simulink model "Cell_Balancer_V_2"  (R2026b)
settings: Solver=VariableStepAuto  StopTime=72000
InitFcn:
  | R=4.2
  | A=.2
  | B=.25
  | C=.24
  | D=.23
  | E=.29
  | F=.22
  | G=.26
  | H=.27
  | I=.28
  | J=.21
libraries: fl_lib x43, nesl_utility x33, batt_lib x10, BatteryCurrentManagement x1
(part 4 of 4)

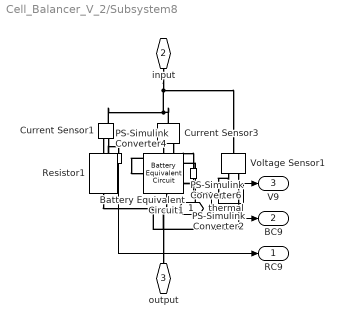
== system Cell_Balancer_V_2/Subsystem8 ==
  Battery Equivalent Circuit1 : batt_lib/Cells/Battery Equivalent Circuit  BatteryCapacity=3 A*hr  ThermalModel=simscape.battery.enum.cells.BatteryThermalModel.LumpedThermalMass  ExtrapolationMethod=simscape.enum.extrapolation.nearest  SOCBreakpoints=[0, .1, .25, .5, .75, .9, 1]  TemperatureBreakpoints=[278, 293, 313] K  OpenCircuitVoltage=[3.5057, 3.566, 3.6337, 3.7127, 3.9259, 4.0777, 4.1928] V  OpenCircuitVoltageThermal=|  VoltageRange=[0, inf] V  HysteresisModel=simscape.battery.enum.cells.HysteresisModel.none  MaximumHysteresisVoltage=[0, 0, 0, 0, 0, 0, 0] V  InstantaneousHysteresisVoltage=[0, 0, 0, 0, 0, 0, 0] V  HysteresisRate=0.1  MaximumHysteresisVoltageThermal=[0, 0, 0; 0, 0, 0; 0, 0, 0; 0, 0, 0; 0, 0, 0; 0, 0, 0; 0, 0, 0] V  InstantaneousHysteresisVoltageThermal=[0, 0, 0; 0, 0, 0; 0, 0, 0; 0, 0, 0; 0, 0, 0; 0, 0, 0; 0, 0, 0] V  HysteresisRateThermal=0.1  ResistanceSOCBreakpoints=[0, .1, .25, .5, .75, .9, 1]  ResistanceTemperatureBreakpoints=[278, 293, 313] K  ResistanceCurrentBreakpoints=[-1, 0, 1] A  CurrentDependence=simscape.battery.enum.cells.CurrentDependence.Disabled  R0=[.0085, .0085, .0087, .0082, .0083, .0085, .0085] Ohm  R0I=[.0117, .0085, .009; .011, .0085, .009; .0114, .0087, .0092; .0107, .0082, .0088; .0107, .0083, .0091; .0113, .0085, .0089; .0116, .0085, .0089] Ohm  R0Thermal=[.0117, .0085, .009; .011, .0085, .009; .0114, .0087, .0092; .0107, .0082, .0088; .0107, .0083, .0091; .0113, .0085, .0089; .0116, .0085, .0089] Ohm  R0ThermalI=repmat([.0117, .0085, .009; .011, .0085, .009; .0114, .0087, .0092; .0107, .0082, .0088; .0107, .0083, .0091; .0113, .0085, .0089; .0116, .0085, .0089], 1, 1, 3) Ohm  DischargeR0=[.0085, .0085, .0087, .0082, .0083, .0085, .0085] Ohm  ChargeR0=[.0085, .0085, .0087, .0082, .0083, .0085, .0085] Ohm  ChargeR0Thermal=[.0117, .0085, .009; .011, .0085, .009; .0114, .0087, .0092; .0107, .0082, .0088; .0107, .0083, .0091; .0113, .0085, .0089; .0116, .0085, .0089] Ohm  DischargeR0Thermal=[.0117, .0085, .009; .011, .0085, .009; .0114, .0087, .0092; .0107, .0082, .0088; .0107, .0083, .0091; .0113, .0085, .0089; .0116, .0085, .0089] Ohm  RCPairs=simscape.battery.enum.cells.RCPairs.noDynamics  R1=[.0029, .0024, .0026, .0016, .0023, .0018, .0017] Ohm  Tau1=[36, 45, 105, 29, 77, 33, 39] s  R2=[.0029, .0024, .0026, .0016, .0023, .0018, .0017] Ohm  Tau2=[36, 45, 105, 29, 77, 33, 39] s  R3=[.0029, .0024, .0026, .0016, .0023, .0018, .0017] Ohm  Tau3=[36, 45, 105, 29, 77, 33, 39] s  R1I=[.0109, .0029, .0013; .0069, .0024, .0012; .0047, .0026, .0013; .0034, .0016, .001; .0033, .0023, .0014; .0033, .0018, .0011; .0028, .0017, .0011] Ohm  Tau1I=[20, 36, 39; 31, 45, 39; 109, 105, 61; 36, 29, 26; 59, 77, 67; 40, 33, 29; 25, 39, 33] s  R2I=[.0109, .0029, .0013; .0069, .0024, .0012; .0047, .0026, .0013; .0034, .0016, .001; .0033, .0023, .0014; .0033, .0018, .0011; .0028, .0017, .0011] Ohm  Tau2I=[20, 36, 39; 31, 45, 39; 109, 105, 61; 36, 29, 26; 59, 77, 67; 40, 33, 29; 25, 39, 33] s  R3I=[.0109, .0029, .0013; .0069, .0024, .0012; .0047, .0026, .0013; .0034, .0016, .001; .0033, .0023, .0014; .0033, .0018, .0011; .0028, .0017, .0011] Ohm  Tau3I=[20, 36, 39; 31, 45, 39; 109, 105, 61; 36, 29, 26; 59, 77, 67; 40, 33, 29; 25, 39, 33] s  DischargeR1=[.0029, .0024, .0026, .0016, .0023, .0018, .0017] Ohm  DischargeTau1=[36, 45, 105, 29, 77, 33, 39] s  ChargeR1=[.0029, .0024, .0026, .0016, .0023, .0018, .0017] Ohm  ChargeTau1=[36, 45, 105, 29, 77, 33, 39] s  DischargeR2=[.0029, .0024, .0026, .0016, .0023, .0018, .0017] Ohm  DischargeTau2=[36, 45, 105, 29, 77, 33, 39] s  ChargeR2=[.0029, .0024, .0026, .0016, .0023, .0018, .0017] Ohm  ChargeTau2=[36, 45, 105, 29, 77, 33, 39] s  DischargeR3=[.0029, .0024, .0026, .0016, .0023, .0018, .0017] Ohm  DischargeTau3=[36, 45, 105, 29, 77, 33, 39] s  ChargeR3=[.0029, .0024, .0026, .0016, .0023, .0018, .0017] Ohm  ChargeTau3=[36, 45, 105, 29, 77, 33, 39] s  R1Thermal=[.0109, .0029, .0013; .0069, .0024, .0012; .0047, .0026, .0013; .0034, .0016, .001; .0033, .0023, .0014; .0033, .0018, .0011; .0028, .0017, .0011] Ohm  Tau1Thermal=[20, 36, 39; 31, 45, 39; 109, 105, 61; 36, 29, 26; 59, 77, 67; 40, 33, 29; 25, 39, 33] s  R2Thermal=[.0109, .0029, .0013; .0069, .0024, .0012; .0047, .0026, .0013; .0034, .0016, .001; .0033, .0023, .0014; .0033, .0018, .0011; .0028, .0017, .0011] Ohm  Tau2Thermal=[20, 36, 39; 31, 45, 39; 109, 105, 61; 36, 29, 26; 59, 77, 67; 40, 33, 29; 25, 39, 33] s  R3Thermal=[.0109, .0029, .0013; .0069, .0024, .0012; .0047, .0026, .0013; .0034, .0016, .001; .0033, .0023, .0014; .0033, .0018, .0011; .0028, .0017, .0011] Ohm  Tau3Thermal=[20, 36, 39; 31, 45, 39; 109, 105, 61; 36, 29, 26; 59, 77, 67; 40, 33, 29; 25, 39, 33] s  R1ThermalI=repmat([.0109, .0029, .0013; .0069, .0024, .0012; .0047, .0026, .0013; .0034, .0016, .001; .0033, .0023, .0014; .0033, .0018, .0011; .0028, .0017, .0011], 1, 1, 3) Ohm  Tau1ThermalI=repmat([20, 36, 39; 31, 45, 39; 109, 105, 61; 36, 29, 26; 59, 77, 67; 40, 33, 29; 25, 39, 33], 1, 1, 3) s  R2ThermalI=repmat([.0109, .0029, .0013; .0069, .0024, .0012; .0047, .0026, .0013; .0034, .0016, .001; .0033, .0023, .0014; .0033, .0018, .0011; .0028, .0017, .0011], 1, 1, 3) Ohm  Tau2ThermalI=repmat([20, 36, 39; 31, 45, 39; 109, 105, 61; 36, 29, 26; 59, 77, 67; 40, 33, 29; 25, 39, 33], 1, 1, 3) s  R3ThermalI=repmat([.0109, .0029, .0013; .0069, .0024, .0012; .0047, .0026, .0013; .0034, .0016, .001; .0033, .0023, .0014; .0033, .0018, .0011; .0028, .0017, .0011], 1, 1, 3) Ohm  Tau3ThermalI=repmat([20, 36, 39; 31, 45, 39; 109, 105, 61; 36, 29, 26; 59, 77, 67; 40, 33, 29; 25, 39, 33], 1, 1, 3) s  DischargeR1Thermal=[.0109, .0029, .0013; .0069, .0024, .0012; .0047, .0026, .0013; .0034, .0016, .001; .0033, .0023, .0014; .0033, .0018, .0011; .0028, .0017, .0011] Ohm  DischargeTau1Thermal=[20, 36, 39; 31, 45, 39; 109, 105, 61; 36, 29, 26; 59, 77, 67; 40, 33, 29; 25, 39, 33] s  ChargeR1Thermal=[.0109, .0029, .0013; .0069, .0024, .0012; .0047, .0026, .0013; .0034, .0016, .001; .0033, .0023, .0014; .0033, .0018, .0011; .0028, .0017, .0011] Ohm  ChargeTau1Thermal=[20, 36, 39; 31, 45, 39; 109, 105, 61; 36, 29, 26; 59, 77, 67; 40, 33, 29; 25, 39, 33] s  DischargeR2Thermal=[.0109, .0029, .0013; .0069, .0024, .0012; .0047, .0026, .0013; .0034, .0016, .001; .0033, .0023, .0014; .0033, .0018, .0011; .0028, .0017, .0011] Ohm  DischargeTau2Thermal=[20, 36, 39; 31, 45, 39; 109, 105, 61; 36, 29, 26; 59, 77, 67; 40, 33, 29; 25, 39, 33] s  ChargeR2Thermal=[.0109, .0029, .0013; .0069, .0024, .0012; .0047, .0026, .0013; .0034, .0016, .001; .0033, .0023, .0014; .0033, .0018, .0011; .0028, .0017, .0011] Ohm  ChargeTau2Thermal=[20, 36, 39; 31, 45, 39; 109, 105, 61; 36, 29, 26; 59, 77, 67; 40, 33, 29; 25, 39, 33] s  DischargeR3Thermal=[.0109, .0029, .0013; .0069, .0024, .0012; .0047, .0026, .0013; .0034, .0016, .001; .0033, .0023, .0014; .0033, .0018, .0011; .0028, .0017, .0011] Ohm  DischargeTau3Thermal=[20, 36, 39; 31, 45, 39; 109, 105, 61; 36, 29, 26; 59, 77, 67; 40, 33, 29; 25, 39, 33] s  ChargeR3Thermal=[.0109, .0029, .0013; .0069, .0024, .0012; .0047, .0026, .0013; .0034, .0016, .001; .0033, .0023, .0014; .0033, .0018, .0011; .0028, .0017, .0011] Ohm  ChargeTau3Thermal=[20, 36, 39; 31, 45, 39; 109, 105, 61; 36, 29, 26; 59, 77, 67; 40, 33, 29; 25, 39, 33] s  SelfDischargeResistor=simscape.battery.enum.cells.BatteryEnable.Disabled  SelfDischargeR=7e3 Ohm  SelfDischargeRThermal=[8000, 7000, 6000] Ohm  CyclingAgingMethod=simscape.battery.enum.cells.CyclingAgingMethod.disabled  CycleCalculationMethod=simscape.battery.enum.cells.CycleCalculationMethod.EquivalentCycles  NumDisCycles=100  OCVChange=0  R0Change=0  CapacityChange=0  SelfDischargeRChange=0  R1Change=0  R2Change=0  R3Change=0  NumDisCyclesBreakpoints=[0, 100, 200, 300]  AgingTemperatureBreakpoints=[298.15, 323.15] K  AgingCurrentBreakpoints=[-.1, -.5, -5] A  OCVChangeVec=[0, 0, 0, 0]  OCVChangeThermal=[0, 0; 0, 0; 0, 0; 0, 0]  R0ChangeVec=[0, 0, 0, 0]  R0ChangeThermal=[0, 0; 0, 0; 0, 0; 0, 0]  R0ChangeThermalI=repmat(0, 4, 2, 3)  R0CyclingChangeInitialTarget=0  CapacityChangeVec=[0, 0, 0, 0]  CapacityChangeThermal=[0, 0; 0, 0; 0, 0; 0, 0]  CapacityChangeThermalI=repmat(0, 4, 2, 3)  CapacityCyclingChangeInitialTarget=0  SelfDischargeRChangeVec=[0, 0, 0, 0]  SelfDischargeRChangeThermal=[0, 0; 0, 0; 0, 0; 0, 0]  SelfDischargeRChangeThermalI=repmat(0, 4, 2, 3)  SelfDischargeRCyclingChangeInitialTarget=0  R1ChangeVec=[0, 0, 0, 0]  R1ChangeThermal=[0, 0; 0, 0; 0, 0; 0, 0]  R1ChangeThermalI=repmat(0, 4, 2, 3)  R1CyclingChangeInitialTarget=0  R2ChangeVec=[0, 0, 0, 0]  R2ChangeThermal=[0, 0; 0, 0; 0, 0; 0, 0]  R2ChangeThermalI=repmat(0, 4, 2, 3)  R2CyclingChangeInitialTarget=0  R3ChangeVec=[0, 0, 0, 0]  R3ChangeThermal=[0, 0; 0, 0; 0, 0; 0, 0]  R3ChangeThermalI=repmat(0, 4, 2, 3)  R3CyclingChangeInitialTarget=0  CalendarAgeResistance=simscape.battery.enum.cells.BatteryEnable.Disabled  CalendarAgeCapacity=simscape.battery.enum.cells.BatteryEnable.Disabled  CalendarAgingMethod=simscape.battery.enum.cells.CalendarAgingMethod.equation  StorageVariable=simscape.battery.enum.cells.StorageVariable.OCV  OCVDuringStorage=0.9  SOCDuringStorage=0.6  StorageTimeIntervals=[0] d  StorageTemperatures=[273] K  ResistanceScalingOCV=2.2134e6  ResistanceScalingOCVOffset=1.632e6  ResistanceExponentialIncrease=0.515833569 V  ResistanceTimeExponent=0.75  ResistanceAgeTemperatureBreakpoints=[273.15, 298.15, 323.15] K  ResistanceAgeTimeBreakpoints=[0, 90, 180, 270] d  PercentResistanceChange=[0, 0, 0]  ResistanceTimeBreakpoints=100 d  PercentResistanceChangeThermal=[0, 0, 0; 0, 0, 0; 0, 0, 0; 0, 0, 0]  CapacityScalingOCV=1.5097e07  CapacityScalingOCVOffset=8.3625e06  CapacityExponentialIncrease=0.6011 V  CapacityTimeExponent=0.75  CapacityAgeTemperatureBreakpoints=[273.15, 298.15, 323.15] K  CapacityAgeTimeBreakpoints=[0, 90, 180, 270] d  PercentCapacityChange=[0, 0, 0]  CapacityTimeBreakpoints=100 d  PercentCapacityChangeThermal=[0, 0, 0; 0, 0, 0; 0, 0, 0; 0, 0, 0]  SimulationTemperature=298.15 K  BatteryThermalMass=100 J/K  NumThermalModels=6  ThermalConductivityZ=18 W/(K*m)  CrossSectionalAreaXY=3.5e-4 m^2  Height=0.07 m  ReversibleHeatModel=simscape.battery.enum.cells.ReversibleHeatModel.Disabled  EntropicCoefficient=[0, 0, 0, 0, 0, 0, 0] mV/K  CurrentDirectionality=simscape.battery.enum.cells.BatteryEnable.Disabled  stateOfCharge_specify=on  stateOfCharge_priority=High  stateOfCharge=I  stateOfCharge_nominal_specify=off  stateOfCharge_nominal_value=1  stateOfCharge_nominal_unit=1  batteryVoltage_specify=off  batteryVoltage_priority=None  batteryVoltage=0 V  batteryVoltage_nominal_specify=off  batteryVoltage_nominal_value=1  batteryVoltage_nominal_unit=V  batteryCurrent_specify=off  batteryCurrent_priority=None  batteryCurrent=0 A  batteryCurrent_nominal_specify=off  batteryCurrent_nominal_value=1  batteryCurrent_nominal_unit=A  numCycles_specify=off  numCycles_priority=High  numCycles=0  numCycles_nominal_specify=off  numCycles_nominal_value=1  numCycles_nominal_unit=1  batteryTemperature_specify=off  batteryTemperature_priority=High  batteryTemperature=298.15 K  batteryTemperature_nominal_specify=off  batteryTemperature_nominal_value=1  batteryTemperature_nominal_unit=K  hysteresisState_specify=off  hysteresisState_priority=High  hysteresisState=0  hysteresisState_nominal_specify=off  hysteresisState_nominal_value=1  hysteresisState_nominal_unit=1  isExothermFaulted_specify=off  isExothermFaulted_priority=None  isExothermFaulted=0  isExothermFaulted_nominal_specify=off  isExothermFaulted_nominal_value=1  isExothermFaulted_nominal_unit=1  reactionHeatRate_specify=off  reactionHeatRate_priority=None  reactionHeatRate=0 W  reactionHeatRate_nominal_specify=off  reactionHeatRate_nominal_value=1  reactionHeatRate_nominal_unit=W  reactionExtent_specify=off  reactionExtent_priority=None  reactionExtent=0  reactionExtent_nominal_specify=off  reactionExtent_nominal_value=1  reactionExtent_nominal_unit=1  shortResistorPower_specify=off  shortResistorPower_priority=None  shortResistorPower=0 W  shortResistorPower_nominal_specify=off  shortResistorPower_nominal_value=1  shortResistorPower_nominal_unit=W
      | [
      |     2.50  2.51  2.52
      |     2.78  2.79  2.80
      |     3.07  3.08  3.09
      |     3.35  3.36  3.37
      |     3.63  3.64  3.65
      |     3.91  3.92  3.93
      |     4.20  4.21  4.22
      | ]
      |  V
  Current Sensor1 : fl_lib/Electrical/Electrical Sensors/Current Sensor
  Current Sensor3 : fl_lib/Electrical/Electrical Sensors/Current Sensor
  PS-Simulink Converter2 : nesl_utility/PS-Simulink Converter  PhysicalDomain=network_engine_domain  SubClassName=ps_output  LeftPortType=input  RightPortType=output  PseudoPeriodic=off  Frequencies=[]  VectorFormat=inherit  Unit=inherit  AffineConversion=off
  PS-Simulink Converter4 : nesl_utility/PS-Simulink Converter  PhysicalDomain=network_engine_domain  SubClassName=ps_output  LeftPortType=input  RightPortType=output  PseudoPeriodic=off  Frequencies=[]  VectorFormat=inherit  Unit=inherit  AffineConversion=off
  PS-Simulink Converter6 : nesl_utility/PS-Simulink Converter  PhysicalDomain=network_engine_domain  SubClassName=ps_output  LeftPortType=input  RightPortType=output  PseudoPeriodic=off  Frequencies=[]  VectorFormat=inherit  Unit=inherit  AffineConversion=off
  Resistor1 : fl_lib/Electrical/Electrical Elements/Resistor  R=R Ohm  i_specify=off  i_priority=None  i=0 A  i_nominal_specify=off  i_nominal_value=1  i_nominal_unit=A  v_specify=off  v_priority=None  v=0 V  v_nominal_specify=off  v_nominal_value=1  v_nominal_unit=V
  Voltage Sensor1 : fl_lib/Electrical/Electrical Sensors/Voltage Sensor
  thermal : PMIOPort  Side=Left
  input : PMIOPort  Port=2  Side=Left
  output : PMIOPort  Port=3  Side=Right
  RC9 : Outport
  BC9 : Outport  Port=2
  V9 : Outport  Port=3
  wires:
  PS-Simulink Converter2/1 -> V9/1
  PS-Simulink Converter4/1 -> RC9/1
  PS-Simulink Converter6/1 -> BC9/1
  connections:
  Battery Equivalent Circuit1/RConn2 -- thermal/RConn1
  Resistor1/RConn1 -- Battery Equivalent Circuit1/RConn1 -- Voltage Sensor1/RConn2 -- output/RConn1
  Current Sensor1/LConn1 -- Current Sensor3/LConn1 -- input/RConn1 -- Voltage Sensor1/LConn1
  Voltage Sensor1/RConn1 -- PS-Simulink Converter2/LConn1
  Current Sensor1/RConn2 -- Resistor1/LConn1
  Current Sensor3/RConn2 -- Battery Equivalent Circuit1/LConn1
  Current Sensor3/RConn1 -- PS-Simulink Converter6/LConn1
  Current Sensor1/RConn1 -- PS-Simulink Converter4/LConn1

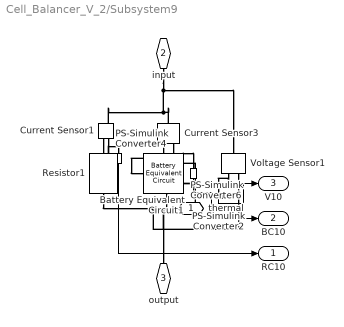
== system Cell_Balancer_V_2/Subsystem9 ==
  Battery Equivalent Circuit1 : batt_lib/Cells/Battery Equivalent Circuit  BatteryCapacity=3 A*hr  ThermalModel=simscape.battery.enum.cells.BatteryThermalModel.LumpedThermalMass  ExtrapolationMethod=simscape.enum.extrapolation.nearest  SOCBreakpoints=[0, .1, .25, .5, .75, .9, 1]  TemperatureBreakpoints=[278, 293, 313] K  OpenCircuitVoltage=[3.5057, 3.566, 3.6337, 3.7127, 3.9259, 4.0777, 4.1928] V  OpenCircuitVoltageThermal=|  VoltageRange=[0, inf] V  HysteresisModel=simscape.battery.enum.cells.HysteresisModel.none  MaximumHysteresisVoltage=[0, 0, 0, 0, 0, 0, 0] V  InstantaneousHysteresisVoltage=[0, 0, 0, 0, 0, 0, 0] V  HysteresisRate=0.1  MaximumHysteresisVoltageThermal=[0, 0, 0; 0, 0, 0; 0, 0, 0; 0, 0, 0; 0, 0, 0; 0, 0, 0; 0, 0, 0] V  InstantaneousHysteresisVoltageThermal=[0, 0, 0; 0, 0, 0; 0, 0, 0; 0, 0, 0; 0, 0, 0; 0, 0, 0; 0, 0, 0] V  HysteresisRateThermal=0.1  ResistanceSOCBreakpoints=[0, .1, .25, .5, .75, .9, 1]  ResistanceTemperatureBreakpoints=[278, 293, 313] K  ResistanceCurrentBreakpoints=[-1, 0, 1] A  CurrentDependence=simscape.battery.enum.cells.CurrentDependence.Disabled  R0=[.0085, .0085, .0087, .0082, .0083, .0085, .0085] Ohm  R0I=[.0117, .0085, .009; .011, .0085, .009; .0114, .0087, .0092; .0107, .0082, .0088; .0107, .0083, .0091; .0113, .0085, .0089; .0116, .0085, .0089] Ohm  R0Thermal=[.0117, .0085, .009; .011, .0085, .009; .0114, .0087, .0092; .0107, .0082, .0088; .0107, .0083, .0091; .0113, .0085, .0089; .0116, .0085, .0089] Ohm  R0ThermalI=repmat([.0117, .0085, .009; .011, .0085, .009; .0114, .0087, .0092; .0107, .0082, .0088; .0107, .0083, .0091; .0113, .0085, .0089; .0116, .0085, .0089], 1, 1, 3) Ohm  DischargeR0=[.0085, .0085, .0087, .0082, .0083, .0085, .0085] Ohm  ChargeR0=[.0085, .0085, .0087, .0082, .0083, .0085, .0085] Ohm  ChargeR0Thermal=[.0117, .0085, .009; .011, .0085, .009; .0114, .0087, .0092; .0107, .0082, .0088; .0107, .0083, .0091; .0113, .0085, .0089; .0116, .0085, .0089] Ohm  DischargeR0Thermal=[.0117, .0085, .009; .011, .0085, .009; .0114, .0087, .0092; .0107, .0082, .0088; .0107, .0083, .0091; .0113, .0085, .0089; .0116, .0085, .0089] Ohm  RCPairs=simscape.battery.enum.cells.RCPairs.noDynamics  R1=[.0029, .0024, .0026, .0016, .0023, .0018, .0017] Ohm  Tau1=[36, 45, 105, 29, 77, 33, 39] s  R2=[.0029, .0024, .0026, .0016, .0023, .0018, .0017] Ohm  Tau2=[36, 45, 105, 29, 77, 33, 39] s  R3=[.0029, .0024, .0026, .0016, .0023, .0018, .0017] Ohm  Tau3=[36, 45, 105, 29, 77, 33, 39] s  R1I=[.0109, .0029, .0013; .0069, .0024, .0012; .0047, .0026, .0013; .0034, .0016, .001; .0033, .0023, .0014; .0033, .0018, .0011; .0028, .0017, .0011] Ohm  Tau1I=[20, 36, 39; 31, 45, 39; 109, 105, 61; 36, 29, 26; 59, 77, 67; 40, 33, 29; 25, 39, 33] s  R2I=[.0109, .0029, .0013; .0069, .0024, .0012; .0047, .0026, .0013; .0034, .0016, .001; .0033, .0023, .0014; .0033, .0018, .0011; .0028, .0017, .0011] Ohm  Tau2I=[20, 36, 39; 31, 45, 39; 109, 105, 61; 36, 29, 26; 59, 77, 67; 40, 33, 29; 25, 39, 33] s  R3I=[.0109, .0029, .0013; .0069, .0024, .0012; .0047, .0026, .0013; .0034, .0016, .001; .0033, .0023, .0014; .0033, .0018, .0011; .0028, .0017, .0011] Ohm  Tau3I=[20, 36, 39; 31, 45, 39; 109, 105, 61; 36, 29, 26; 59, 77, 67; 40, 33, 29; 25, 39, 33] s  DischargeR1=[.0029, .0024, .0026, .0016, .0023, .0018, .0017] Ohm  DischargeTau1=[36, 45, 105, 29, 77, 33, 39] s  ChargeR1=[.0029, .0024, .0026, .0016, .0023, .0018, .0017] Ohm  ChargeTau1=[36, 45, 105, 29, 77, 33, 39] s  DischargeR2=[.0029, .0024, .0026, .0016, .0023, .0018, .0017] Ohm  DischargeTau2=[36, 45, 105, 29, 77, 33, 39] s  ChargeR2=[.0029, .0024, .0026, .0016, .0023, .0018, .0017] Ohm  ChargeTau2=[36, 45, 105, 29, 77, 33, 39] s  DischargeR3=[.0029, .0024, .0026, .0016, .0023, .0018, .0017] Ohm  DischargeTau3=[36, 45, 105, 29, 77, 33, 39] s  ChargeR3=[.0029, .0024, .0026, .0016, .0023, .0018, .0017] Ohm  ChargeTau3=[36, 45, 105, 29, 77, 33, 39] s  R1Thermal=[.0109, .0029, .0013; .0069, .0024, .0012; .0047, .0026, .0013; .0034, .0016, .001; .0033, .0023, .0014; .0033, .0018, .0011; .0028, .0017, .0011] Ohm  Tau1Thermal=[20, 36, 39; 31, 45, 39; 109, 105, 61; 36, 29, 26; 59, 77, 67; 40, 33, 29; 25, 39, 33] s  R2Thermal=[.0109, .0029, .0013; .0069, .0024, .0012; .0047, .0026, .0013; .0034, .0016, .001; .0033, .0023, .0014; .0033, .0018, .0011; .0028, .0017, .0011] Ohm  Tau2Thermal=[20, 36, 39; 31, 45, 39; 109, 105, 61; 36, 29, 26; 59, 77, 67; 40, 33, 29; 25, 39, 33] s  R3Thermal=[.0109, .0029, .0013; .0069, .0024, .0012; .0047, .0026, .0013; .0034, .0016, .001; .0033, .0023, .0014; .0033, .0018, .0011; .0028, .0017, .0011] Ohm  Tau3Thermal=[20, 36, 39; 31, 45, 39; 109, 105, 61; 36, 29, 26; 59, 77, 67; 40, 33, 29; 25, 39, 33] s  R1ThermalI=repmat([.0109, .0029, .0013; .0069, .0024, .0012; .0047, .0026, .0013; .0034, .0016, .001; .0033, .0023, .0014; .0033, .0018, .0011; .0028, .0017, .0011], 1, 1, 3) Ohm  Tau1ThermalI=repmat([20, 36, 39; 31, 45, 39; 109, 105, 61; 36, 29, 26; 59, 77, 67; 40, 33, 29; 25, 39, 33], 1, 1, 3) s  R2ThermalI=repmat([.0109, .0029, .0013; .0069, .0024, .0012; .0047, .0026, .0013; .0034, .0016, .001; .0033, .0023, .0014; .0033, .0018, .0011; .0028, .0017, .0011], 1, 1, 3) Ohm  Tau2ThermalI=repmat([20, 36, 39; 31, 45, 39; 109, 105, 61; 36, 29, 26; 59, 77, 67; 40, 33, 29; 25, 39, 33], 1, 1, 3) s  R3ThermalI=repmat([.0109, .0029, .0013; .0069, .0024, .0012; .0047, .0026, .0013; .0034, .0016, .001; .0033, .0023, .0014; .0033, .0018, .0011; .0028, .0017, .0011], 1, 1, 3) Ohm  Tau3ThermalI=repmat([20, 36, 39; 31, 45, 39; 109, 105, 61; 36, 29, 26; 59, 77, 67; 40, 33, 29; 25, 39, 33], 1, 1, 3) s  DischargeR1Thermal=[.0109, .0029, .0013; .0069, .0024, .0012; .0047, .0026, .0013; .0034, .0016, .001; .0033, .0023, .0014; .0033, .0018, .0011; .0028, .0017, .0011] Ohm  DischargeTau1Thermal=[20, 36, 39; 31, 45, 39; 109, 105, 61; 36, 29, 26; 59, 77, 67; 40, 33, 29; 25, 39, 33] s  ChargeR1Thermal=[.0109, .0029, .0013; .0069, .0024, .0012; .0047, .0026, .0013; .0034, .0016, .001; .0033, .0023, .0014; .0033, .0018, .0011; .0028, .0017, .0011] Ohm  ChargeTau1Thermal=[20, 36, 39; 31, 45, 39; 109, 105, 61; 36, 29, 26; 59, 77, 67; 40, 33, 29; 25, 39, 33] s  DischargeR2Thermal=[.0109, .0029, .0013; .0069, .0024, .0012; .0047, .0026, .0013; .0034, .0016, .001; .0033, .0023, .0014; .0033, .0018, .0011; .0028, .0017, .0011] Ohm  DischargeTau2Thermal=[20, 36, 39; 31, 45, 39; 109, 105, 61; 36, 29, 26; 59, 77, 67; 40, 33, 29; 25, 39, 33] s  ChargeR2Thermal=[.0109, .0029, .0013; .0069, .0024, .0012; .0047, .0026, .0013; .0034, .0016, .001; .0033, .0023, .0014; .0033, .0018, .0011; .0028, .0017, .0011] Ohm  ChargeTau2Thermal=[20, 36, 39; 31, 45, 39; 109, 105, 61; 36, 29, 26; 59, 77, 67; 40, 33, 29; 25, 39, 33] s  DischargeR3Thermal=[.0109, .0029, .0013; .0069, .0024, .0012; .0047, .0026, .0013; .0034, .0016, .001; .0033, .0023, .0014; .0033, .0018, .0011; .0028, .0017, .0011] Ohm  DischargeTau3Thermal=[20, 36, 39; 31, 45, 39; 109, 105, 61; 36, 29, 26; 59, 77, 67; 40, 33, 29; 25, 39, 33] s  ChargeR3Thermal=[.0109, .0029, .0013; .0069, .0024, .0012; .0047, .0026, .0013; .0034, .0016, .001; .0033, .0023, .0014; .0033, .0018, .0011; .0028, .0017, .0011] Ohm  ChargeTau3Thermal=[20, 36, 39; 31, 45, 39; 109, 105, 61; 36, 29, 26; 59, 77, 67; 40, 33, 29; 25, 39, 33] s  SelfDischargeResistor=simscape.battery.enum.cells.BatteryEnable.Disabled  SelfDischargeR=7e3 Ohm  SelfDischargeRThermal=[8000, 7000, 6000] Ohm  CyclingAgingMethod=simscape.battery.enum.cells.CyclingAgingMethod.disabled  CycleCalculationMethod=simscape.battery.enum.cells.CycleCalculationMethod.EquivalentCycles  NumDisCycles=100  OCVChange=0  R0Change=0  CapacityChange=0  SelfDischargeRChange=0  R1Change=0  R2Change=0  R3Change=0  NumDisCyclesBreakpoints=[0, 100, 200, 300]  AgingTemperatureBreakpoints=[298.15, 323.15] K  AgingCurrentBreakpoints=[-.1, -.5, -5] A  OCVChangeVec=[0, 0, 0, 0]  OCVChangeThermal=[0, 0; 0, 0; 0, 0; 0, 0]  R0ChangeVec=[0, 0, 0, 0]  R0ChangeThermal=[0, 0; 0, 0; 0, 0; 0, 0]  R0ChangeThermalI=repmat(0, 4, 2, 3)  R0CyclingChangeInitialTarget=0  CapacityChangeVec=[0, 0, 0, 0]  CapacityChangeThermal=[0, 0; 0, 0; 0, 0; 0, 0]  CapacityChangeThermalI=repmat(0, 4, 2, 3)  CapacityCyclingChangeInitialTarget=0  SelfDischargeRChangeVec=[0, 0, 0, 0]  SelfDischargeRChangeThermal=[0, 0; 0, 0; 0, 0; 0, 0]  SelfDischargeRChangeThermalI=repmat(0, 4, 2, 3)  SelfDischargeRCyclingChangeInitialTarget=0  R1ChangeVec=[0, 0, 0, 0]  R1ChangeThermal=[0, 0; 0, 0; 0, 0; 0, 0]  R1ChangeThermalI=repmat(0, 4, 2, 3)  R1CyclingChangeInitialTarget=0  R2ChangeVec=[0, 0, 0, 0]  R2ChangeThermal=[0, 0; 0, 0; 0, 0; 0, 0]  R2ChangeThermalI=repmat(0, 4, 2, 3)  R2CyclingChangeInitialTarget=0  R3ChangeVec=[0, 0, 0, 0]  R3ChangeThermal=[0, 0; 0, 0; 0, 0; 0, 0]  R3ChangeThermalI=repmat(0, 4, 2, 3)  R3CyclingChangeInitialTarget=0  CalendarAgeResistance=simscape.battery.enum.cells.BatteryEnable.Disabled  CalendarAgeCapacity=simscape.battery.enum.cells.BatteryEnable.Disabled  CalendarAgingMethod=simscape.battery.enum.cells.CalendarAgingMethod.equation  StorageVariable=simscape.battery.enum.cells.StorageVariable.OCV  OCVDuringStorage=0.9  SOCDuringStorage=0.6  StorageTimeIntervals=[0] d  StorageTemperatures=[273] K  ResistanceScalingOCV=2.2134e6  ResistanceScalingOCVOffset=1.632e6  ResistanceExponentialIncrease=0.515833569 V  ResistanceTimeExponent=0.75  ResistanceAgeTemperatureBreakpoints=[273.15, 298.15, 323.15] K  ResistanceAgeTimeBreakpoints=[0, 90, 180, 270] d  PercentResistanceChange=[0, 0, 0]  ResistanceTimeBreakpoints=100 d  PercentResistanceChangeThermal=[0, 0, 0; 0, 0, 0; 0, 0, 0; 0, 0, 0]  CapacityScalingOCV=1.5097e07  CapacityScalingOCVOffset=8.3625e06  CapacityExponentialIncrease=0.6011 V  CapacityTimeExponent=0.75  CapacityAgeTemperatureBreakpoints=[273.15, 298.15, 323.15] K  CapacityAgeTimeBreakpoints=[0, 90, 180, 270] d  PercentCapacityChange=[0, 0, 0]  CapacityTimeBreakpoints=100 d  PercentCapacityChangeThermal=[0, 0, 0; 0, 0, 0; 0, 0, 0; 0, 0, 0]  SimulationTemperature=298.15 K  BatteryThermalMass=100 J/K  NumThermalModels=6  ThermalConductivityZ=18 W/(K*m)  CrossSectionalAreaXY=3.5e-4 m^2  Height=0.07 m  ReversibleHeatModel=simscape.battery.enum.cells.ReversibleHeatModel.Disabled  EntropicCoefficient=[0, 0, 0, 0, 0, 0, 0] mV/K  CurrentDirectionality=simscape.battery.enum.cells.BatteryEnable.Disabled  stateOfCharge_specify=on  stateOfCharge_priority=High  stateOfCharge=J  stateOfCharge_nominal_specify=off  stateOfCharge_nominal_value=1  stateOfCharge_nominal_unit=1  batteryVoltage_specify=off  batteryVoltage_priority=None  batteryVoltage=0 V  batteryVoltage_nominal_specify=off  batteryVoltage_nominal_value=1  batteryVoltage_nominal_unit=V  batteryCurrent_specify=off  batteryCurrent_priority=None  batteryCurrent=0 A  batteryCurrent_nominal_specify=off  batteryCurrent_nominal_value=1  batteryCurrent_nominal_unit=A  numCycles_specify=off  numCycles_priority=High  numCycles=0  numCycles_nominal_specify=off  numCycles_nominal_value=1  numCycles_nominal_unit=1  batteryTemperature_specify=off  batteryTemperature_priority=High  batteryTemperature=298.15 K  batteryTemperature_nominal_specify=off  batteryTemperature_nominal_value=1  batteryTemperature_nominal_unit=K  hysteresisState_specify=off  hysteresisState_priority=High  hysteresisState=0  hysteresisState_nominal_specify=off  hysteresisState_nominal_value=1  hysteresisState_nominal_unit=1  isExothermFaulted_specify=off  isExothermFaulted_priority=None  isExothermFaulted=0  isExothermFaulted_nominal_specify=off  isExothermFaulted_nominal_value=1  isExothermFaulted_nominal_unit=1  reactionHeatRate_specify=off  reactionHeatRate_priority=None  reactionHeatRate=0 W  reactionHeatRate_nominal_specify=off  reactionHeatRate_nominal_value=1  reactionHeatRate_nominal_unit=W  reactionExtent_specify=off  reactionExtent_priority=None  reactionExtent=0  reactionExtent_nominal_specify=off  reactionExtent_nominal_value=1  reactionExtent_nominal_unit=1  shortResistorPower_specify=off  shortResistorPower_priority=None  shortResistorPower=0 W  shortResistorPower_nominal_specify=off  shortResistorPower_nominal_value=1  shortResistorPower_nominal_unit=W
      | [
      |     2.50  2.51  2.52
      |     2.78  2.79  2.80
      |     3.07  3.08  3.09
      |     3.35  3.36  3.37
      |     3.63  3.64  3.65
      |     3.91  3.92  3.93
      |     4.20  4.21  4.22
      | ]
      |  V
  Current Sensor1 : fl_lib/Electrical/Electrical Sensors/Current Sensor
  Current Sensor3 : fl_lib/Electrical/Electrical Sensors/Current Sensor
  PS-Simulink Converter2 : nesl_utility/PS-Simulink Converter  PhysicalDomain=network_engine_domain  SubClassName=ps_output  LeftPortType=input  RightPortType=output  PseudoPeriodic=off  Frequencies=[]  VectorFormat=inherit  Unit=inherit  AffineConversion=off
  PS-Simulink Converter4 : nesl_utility/PS-Simulink Converter  PhysicalDomain=network_engine_domain  SubClassName=ps_output  LeftPortType=input  RightPortType=output  PseudoPeriodic=off  Frequencies=[]  VectorFormat=inherit  Unit=inherit  AffineConversion=off
  PS-Simulink Converter6 : nesl_utility/PS-Simulink Converter  PhysicalDomain=network_engine_domain  SubClassName=ps_output  LeftPortType=input  RightPortType=output  PseudoPeriodic=off  Frequencies=[]  VectorFormat=inherit  Unit=inherit  AffineConversion=off
  Resistor1 : fl_lib/Electrical/Electrical Elements/Resistor  R=R Ohm  i_specify=off  i_priority=None  i=0 A  i_nominal_specify=off  i_nominal_value=1  i_nominal_unit=A  v_specify=off  v_priority=None  v=0 V  v_nominal_specify=off  v_nominal_value=1  v_nominal_unit=V
  Voltage Sensor1 : fl_lib/Electrical/Electrical Sensors/Voltage Sensor
  thermal : PMIOPort  Side=Left
  input : PMIOPort  Port=2  Side=Left
  output : PMIOPort  Port=3  Side=Right
  RC10 : Outport
  BC10 : Outport  Port=2
  V10 : Outport  Port=3
  wires:
  PS-Simulink Converter2/1 -> V10/1
  PS-Simulink Converter4/1 -> RC10/1
  PS-Simulink Converter6/1 -> BC10/1
  connections:
  Battery Equivalent Circuit1/RConn2 -- thermal/RConn1
  Resistor1/RConn1 -- Battery Equivalent Circuit1/RConn1 -- Voltage Sensor1/RConn2 -- output/RConn1
  Current Sensor1/LConn1 -- Current Sensor3/LConn1 -- input/RConn1 -- Voltage Sensor1/LConn1
  Voltage Sensor1/RConn1 -- PS-Simulink Converter2/LConn1
  Current Sensor1/RConn2 -- Resistor1/LConn1
  Current Sensor3/RConn2 -- Battery Equivalent Circuit1/LConn1
  Current Sensor3/RConn1 -- PS-Simulink Converter6/LConn1
  Current Sensor1/RConn1 -- PS-Simulink Converter4/LConn1
